simulink model "test_LQI_z"  (R2025b)
settings: Solver=FixedStepAuto  StartTime=0.0  StopTime=10  FixedStep=0.05  RelTol=1e-3
values from neighbouring files (symbols this model uses):
  Kd = 0.8 * K_aug(2)    [gains_LQI.m]
  Ki = 0.8 * K_aug(3)    [gains_LQI.m]
  Kp = 0.8 * K_aug(1)    [gains_LQI.m]
  tau = 1.2    [gains_LQI.m]
undefined symbols (not defined in the file or in its folder): DiscIntNeverNeededParam
settings Model: Creator=anoua  LastModifiedBy=anoua

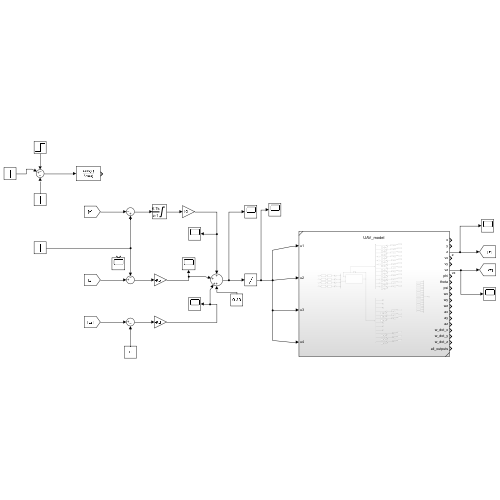
[thumbnail: Simulink's stored preview of the top-level diagram]
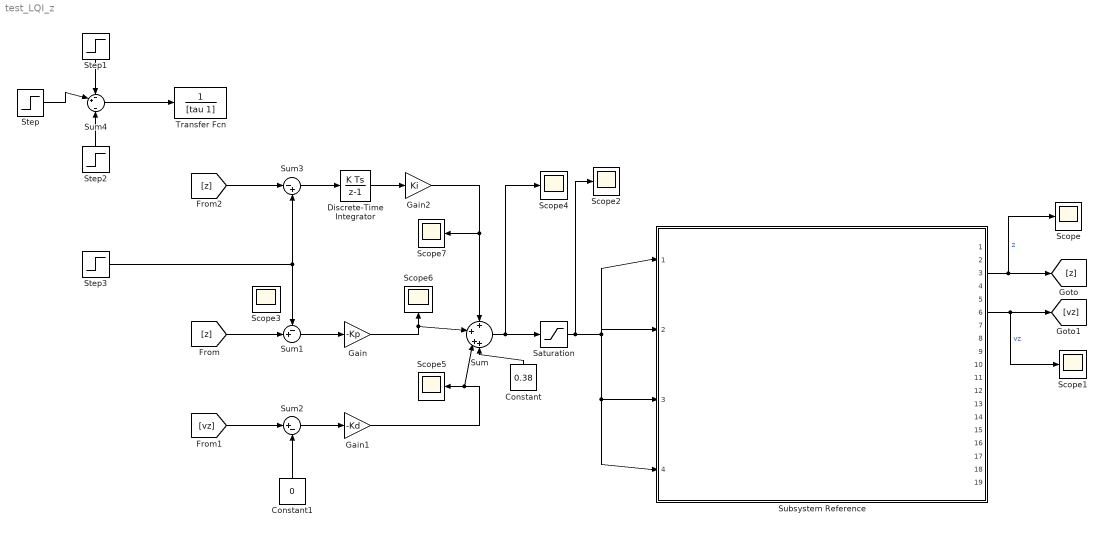
== system test_LQI_z ==
  Constant : Constant  Value=0.38
  Constant1 : Constant  Value=0
  Discrete-Time Integrator : DiscreteIntegrator  SampleTime=-1  LimitOutput=on  UpperSaturationLimit=1/Ki  LowerSaturationLimit=-1/Ki  ICPrevOutput=DiscIntNeverNeededParam  ICPrevScaledInput=DiscIntNeverNeededParam
  Gain : Gain  Gain=-Kp
  Gain1 : Gain  Gain=-Kd
  Gain2 : Gain  Gain=Ki
  Saturation : Saturate  UpperLimit=1  LowerLimit=-1
  Scope{,1..7} (8 alike) : Scope
      Scope settings: ActiveDisplayYMinimum=-0.1837823327602342  ActiveDisplayYMaximum=0.50285338455195117
      Scope1 settings: ActiveDisplayYMinimum=-1.3340291702690279  ActiveDisplayYMaximum=1.1408884147091976
      Scope2 settings: ActiveDisplayYMinimum=-0.21929507601178058  ActiveDisplayYMaximum=1.1354772306679757  DataLoggingVariableName=ScopeData2
      Scope3 settings: ActiveDisplayYMinimum=-0.53484809981403014  ActiveDisplayYMaximum=1.6271171549271228  DataLoggingVariableName=ScopeData3
      Scope4 settings: ActiveDisplayYMinimum=-0.20597858411759526  ActiveDisplayYMaximum=1.3433393659109518  DataLoggingVariableName=ScopeData4
      Scope5 settings: ActiveDisplayYMinimum=-1.1589224197542392  ActiveDisplayYMaximum=1.1177428824029849  DataLoggingVariableName=ScopeData5
      Scope6 settings: ActiveDisplayYMinimum=-0.255322559757432  ActiveDisplayYMaximum=1.4597245843788387  DataLoggingVariableName=ScopeData6
      Scope7 settings: ActiveDisplayYMinimum=-0.0942981106684779  ActiveDisplayYMaximum=0.45559235947762056  DataLoggingVariableName=ScopeData7
  Step : Step  Time=0  After=0.5  SampleTime=0
  Step1 : Step  Time=12  After=0.65  SampleTime=0
  Step2 : Step  Time=16  After=0.1  SampleTime=0
  Step3 : Step  Time=5  After=0.5  SampleTime=0
  Subsystem Reference : Subsystem  ReferencedSubsystem=UAV_model
  Sum : Sum  Inputs=+|+|++
  Sum1 : Sum  Inputs=-+|
  Sum2 : Sum  Inputs=|+-
  Sum3 : Sum  Inputs=|-+
  Sum4 : Sum  Inputs=-+|-
  Transfer Fcn : TransferFcn  Denominator=[tau 1]
  wires:
  Subsystem Reference/3 -> [z], Scope/1  "z"
  [z] -> Sum1/2
  Sum1/1 -> Gain/1
  Subsystem Reference/6 -> [vz], Scope1/1  "vz"
  [vz] -> Sum2/1
  Constant1/1 -> Sum2/2
  Sum2/1 -> Gain1/1
  Gain/1 -> Scope6/1, Sum/2
  Gain1/1 -> Sum/3, Scope5/1
  [z] -> Sum3/1
  Gain2/1 -> Scope7/1, Sum/1
  Sum/1 -> Scope4/1, Saturation/1
  Saturation/1 -> Subsystem Reference/1, Subsystem Reference/2, Subsystem Reference/4, Subsystem Reference/3, Scope2/1
  Sum3/1 -> Discrete-Time Integrator/1
  Discrete-Time Integrator/1 -> Gain2/1
  Step/1 -> Sum4/2
  Step1/1 -> Sum4/1
  Sum4/1 -> Transfer Fcn/1
  Constant/1 -> Sum/4
  Step2/1 -> Sum4/3
  Step3/1 -> Sum3/2, Sum1/1
